simulink model "EmfObserver"  (R2026b)
settings: Solver=VariableStepAuto
undefined symbols (not defined in the file or in its folder): emfCfg, pllCfg
libraries: AngleTracking x2
settings Model: Creator=24322  LastModifiedBy=24322

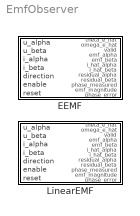
== system EmfObserver ==
  EEMF : Subsystem  mask{cfg=emfCfg, trackerCfg=pllCfg}
      mask prompts: cfg "Observer configuration"; trackerCfg "PLL configuration"
  LinearEMF : Subsystem  mask{cfg=emfCfg, trackerCfg=pllCfg}
      mask prompts: cfg "Observer configuration"; trackerCfg "PLL configuration"

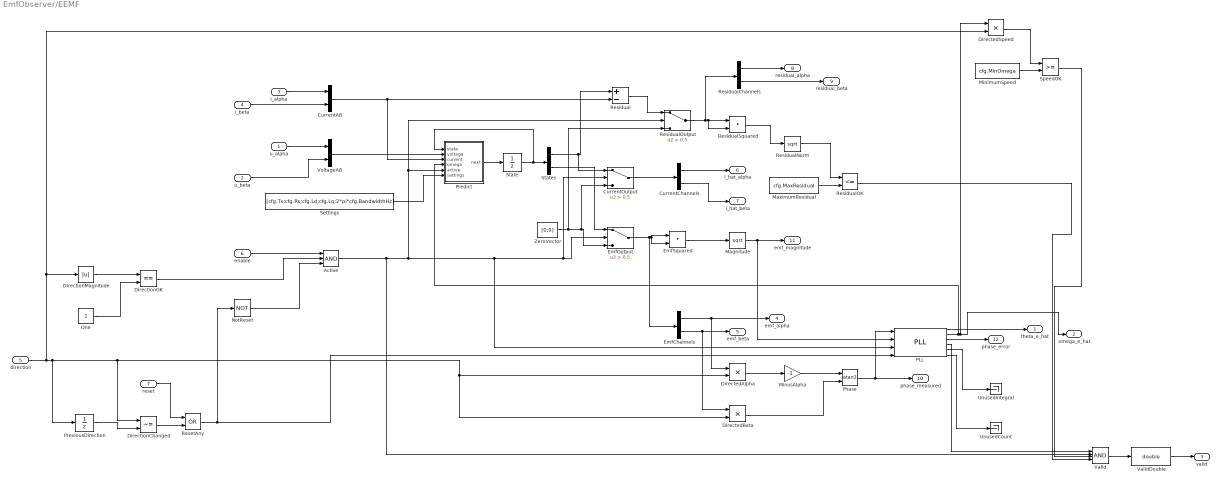
== system EmfObserver/EEMF ==
  u_alpha : Inport  SampleTime=cfg.Ts
  u_beta : Inport  Port=2  SampleTime=cfg.Ts
  i_alpha : Inport  Port=3  SampleTime=cfg.Ts
  i_beta : Inport  Port=4  SampleTime=cfg.Ts
  direction : Inport  Port=5  SampleTime=cfg.Ts
  enable : Inport  Port=6  SampleTime=cfg.Ts
  reset : Inport  Port=7  SampleTime=cfg.Ts
  Active : Logic  Inputs=3  IconShape=distinctive  AllPortsSameDT=off  OutDataTypeStr=boolean
  CurrentAB : Mux  Inputs=2
  CurrentChannels : Demux  Outputs=2
  CurrentOutput : Switch  Criteria=u2 > Threshold  Threshold=0.5  SaturateOnIntegerOverflow=off  InputSameDT=off
  DirectedAlpha : Product  Inputs=**
  DirectedBeta : Product  Inputs=**
  DirectedSpeed : Product  Inputs=**
  DirectionChanged : RelationalOperator  Operator=~=  OutDataTypeStr=boolean  RndMeth=Simplest  InputSameDT=off
  DirectionMagnitude : Abs  SaturateOnIntegerOverflow=off
  DirectionOK : RelationalOperator  Operator===  OutDataTypeStr=boolean  RndMeth=Simplest  InputSameDT=off
  EmfChannels : Demux  Outputs=2
  EmfOutput : Switch  Criteria=u2 > Threshold  Threshold=0.5  SaturateOnIntegerOverflow=off  InputSameDT=off
  EmfSquared : DotProduct  OutDataTypeStr=Inherit: Inherit via internal rule
  Magnitude : Sqrt
  MaximumResidual : Constant  Value=cfg.MaxResidual
  MinimumSpeed : Constant  Value=cfg.MinOmega
  MinusAlpha : Gain  Gain=-1
  NotReset : Logic  Operator=NOT  IconShape=distinctive  AllPortsSameDT=off  OutDataTypeStr=boolean
  One : Constant
  PLL : AngleTracking/PLL  pllCfg=trackerCfg
  Phase : Trigonometry  Operator=atan2
  Predict : MATLAB Function  TreatAsAtomicUnit=on
  PreviousDirection : UnitDelay  SampleTime=cfg.Ts
  ResetAny : Logic  Operator=OR  IconShape=distinctive  AllPortsSameDT=off  OutDataTypeStr=boolean
  Residual : Sum  Inputs=+-
  ResidualChannels : Demux  Outputs=2
  ResidualNorm : Sqrt
  ResidualOK : RelationalOperator  Operator=<=  OutDataTypeStr=boolean  RndMeth=Simplest  InputSameDT=off
  ResidualOutput : Switch  Criteria=u2 > Threshold  Threshold=0.5  SaturateOnIntegerOverflow=off  InputSameDT=off
  ResidualSquared : DotProduct  OutDataTypeStr=Inherit: Inherit via internal rule
  Settings : Constant  Value=[cfg.Ts;cfg.Rs;cfg.Ld;cfg.Lq;2*pi*cfg.BandwidthHz]
  SpeedOK : RelationalOperator  OutDataTypeStr=boolean  RndMeth=Simplest  InputSameDT=off
  State : UnitDelay  InitialCondition=zeros(4,1)  SampleTime=cfg.Ts
  States : Demux  Outputs=2
  UnusedCount : Terminator
  UnusedIntegral : Terminator
  Valid : Logic  Inputs=4  IconShape=distinctive  AllPortsSameDT=off  OutDataTypeStr=boolean
  ValidDouble : DataTypeConversion  OutDataTypeStr=double  SaturateOnIntegerOverflow=off  RndMeth=Floor
  VoltageAB : Mux  Inputs=2
  ZeroVector : Constant  Value=[0;0]
  theta_e_hat : Outport
  omega_e_hat : Outport  Port=2
  valid : Outport  Port=3
  emf_alpha : Outport  Port=4
  emf_beta : Outport  Port=5
  i_hat_alpha : Outport  Port=6
  i_hat_beta : Outport  Port=7
  residual_alpha : Outport  Port=8
  residual_beta : Outport  Port=9
  phase_measured : Outport  Port=10
  emf_magnitude : Outport  Port=11
  phase_error : Outport  Port=12
  wires:
  ResidualChannels/2 -> residual_beta/1
  CurrentChannels/2 -> i_hat_beta/1
  ResidualChannels/1 -> residual_alpha/1
  CurrentChannels/1 -> i_hat_alpha/1
  PLL/6 -> UnusedCount/1
  PLL/5 -> UnusedIntegral/1
  PLL/4 -> Valid/1
  PLL/3 -> phase_error/1
  PLL/1 -> theta_e_hat/1
  EmfChannels/2 -> emf_beta/1, DirectedBeta/1
  EmfChannels/1 -> emf_alpha/1, DirectedAlpha/1
  States/2 -> EmfOutput/1
  States/1 -> CurrentOutput/1, Residual/1
  Predict/1(next) -> State/1
  Settings/1 -> Predict/6(settings)
  PLL/2 -> omega_e_hat/1, DirectedSpeed/1, Predict/4(omega)
  VoltageAB/1 -> Predict/2(voltage)
  ValidDouble/1 -> valid/1
  Valid/1 -> ValidDouble/1
  ResidualOK/1 -> Valid/4
  SpeedOK/1 -> Valid/3
  MinimumSpeed/1 -> SpeedOK/2
  DirectedSpeed/1 -> SpeedOK/1
  Magnitude/1 -> PLL/2, emf_magnitude/1
  Phase/1 -> PLL/1, phase_measured/1
  DirectedBeta/1 -> Phase/2
  MinusAlpha/1 -> Phase/1
  DirectedAlpha/1 -> MinusAlpha/1
  EmfSquared/1 -> Magnitude/1
  MaximumResidual/1 -> ResidualOK/2
  ResidualNorm/1 -> ResidualOK/1
  ResidualSquared/1 -> ResidualNorm/1
  ZeroVector/1 -> CurrentOutput/3, EmfOutput/3, ResidualOutput/3
  Active/1 -> CurrentOutput/2, EmfOutput/2, PLL/3, ResidualOutput/2, Predict/5(active), Valid/2
  Residual/1 -> ResidualOutput/1
  CurrentAB/1 -> Residual/2, Predict/3(current)
  ResidualOutput/1 -> ResidualSquared/1, ResidualSquared/2, ResidualChannels/1
  EmfOutput/1 -> EmfSquared/1, EmfSquared/2, EmfChannels/1
  CurrentOutput/1 -> CurrentChannels/1
  State/1 -> States/1, Predict/1(state)
  NotReset/1 -> Active/3
  DirectionOK/1 -> Active/2
  enable/1 -> Active/1
  ResetAny/1 -> NotReset/1, PLL/4
  DirectionChanged/1 -> ResetAny/2
  reset/1 -> ResetAny/1
  PreviousDirection/1 -> DirectionChanged/2
  One/1 -> DirectionOK/2
  DirectionMagnitude/1 -> DirectionOK/1
  direction/1 -> DirectedAlpha/2, DirectedBeta/2, DirectionChanged/1, PreviousDirection/1, DirectionMagnitude/1, DirectedSpeed/2
  i_beta/1 -> CurrentAB/2
  i_alpha/1 -> CurrentAB/1
  u_beta/1 -> VoltageAB/2
  u_alpha/1 -> VoltageAB/1

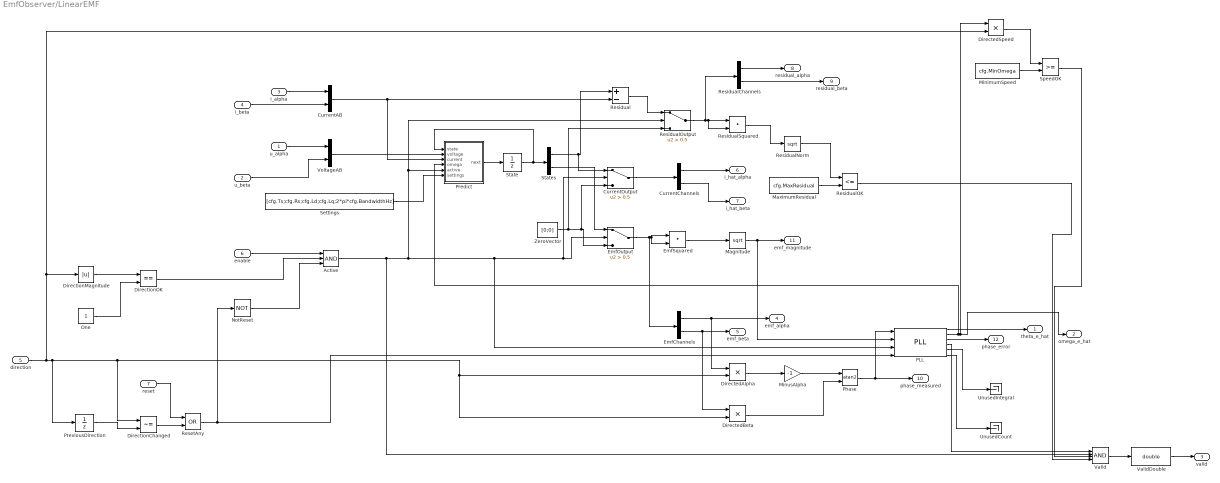
== system EmfObserver/LinearEMF ==
  u_alpha : Inport  SampleTime=cfg.Ts
  u_beta : Inport  Port=2  SampleTime=cfg.Ts
  i_alpha : Inport  Port=3  SampleTime=cfg.Ts
  i_beta : Inport  Port=4  SampleTime=cfg.Ts
  direction : Inport  Port=5  SampleTime=cfg.Ts
  enable : Inport  Port=6  SampleTime=cfg.Ts
  reset : Inport  Port=7  SampleTime=cfg.Ts
  Active : Logic  Inputs=3  IconShape=distinctive  AllPortsSameDT=off  OutDataTypeStr=boolean
  CurrentAB : Mux  Inputs=2
  CurrentChannels : Demux  Outputs=2
  CurrentOutput : Switch  Criteria=u2 > Threshold  Threshold=0.5  SaturateOnIntegerOverflow=off  InputSameDT=off
  DirectedAlpha : Product  Inputs=**
  DirectedBeta : Product  Inputs=**
  DirectedSpeed : Product  Inputs=**
  DirectionChanged : RelationalOperator  Operator=~=  OutDataTypeStr=boolean  RndMeth=Simplest  InputSameDT=off
  DirectionMagnitude : Abs  SaturateOnIntegerOverflow=off
  DirectionOK : RelationalOperator  Operator===  OutDataTypeStr=boolean  RndMeth=Simplest  InputSameDT=off
  EmfChannels : Demux  Outputs=2
  EmfOutput : Switch  Criteria=u2 > Threshold  Threshold=0.5  SaturateOnIntegerOverflow=off  InputSameDT=off
  EmfSquared : DotProduct  OutDataTypeStr=Inherit: Inherit via internal rule
  Magnitude : Sqrt
  MaximumResidual : Constant  Value=cfg.MaxResidual
  MinimumSpeed : Constant  Value=cfg.MinOmega
  MinusAlpha : Gain  Gain=-1
  NotReset : Logic  Operator=NOT  IconShape=distinctive  AllPortsSameDT=off  OutDataTypeStr=boolean
  One : Constant
  PLL : AngleTracking/PLL  pllCfg=trackerCfg
  Phase : Trigonometry  Operator=atan2
  Predict : MATLAB Function  TreatAsAtomicUnit=on
  PreviousDirection : UnitDelay  SampleTime=cfg.Ts
  ResetAny : Logic  Operator=OR  IconShape=distinctive  AllPortsSameDT=off  OutDataTypeStr=boolean
  Residual : Sum  Inputs=+-
  ResidualChannels : Demux  Outputs=2
  ResidualNorm : Sqrt
  ResidualOK : RelationalOperator  Operator=<=  OutDataTypeStr=boolean  RndMeth=Simplest  InputSameDT=off
  ResidualOutput : Switch  Criteria=u2 > Threshold  Threshold=0.5  SaturateOnIntegerOverflow=off  InputSameDT=off
  ResidualSquared : DotProduct  OutDataTypeStr=Inherit: Inherit via internal rule
  Settings : Constant  Value=[cfg.Ts;cfg.Rs;cfg.Ld;cfg.Lq;2*pi*cfg.BandwidthHz]
  SpeedOK : RelationalOperator  OutDataTypeStr=boolean  RndMeth=Simplest  InputSameDT=off
  State : UnitDelay  InitialCondition=zeros(4,1)  SampleTime=cfg.Ts
  States : Demux  Outputs=2
  UnusedCount : Terminator
  UnusedIntegral : Terminator
  Valid : Logic  Inputs=4  IconShape=distinctive  AllPortsSameDT=off  OutDataTypeStr=boolean
  ValidDouble : DataTypeConversion  OutDataTypeStr=double  SaturateOnIntegerOverflow=off  RndMeth=Floor
  VoltageAB : Mux  Inputs=2
  ZeroVector : Constant  Value=[0;0]
  theta_e_hat : Outport
  omega_e_hat : Outport  Port=2
  valid : Outport  Port=3
  emf_alpha : Outport  Port=4
  emf_beta : Outport  Port=5
  i_hat_alpha : Outport  Port=6
  i_hat_beta : Outport  Port=7
  residual_alpha : Outport  Port=8
  residual_beta : Outport  Port=9
  phase_measured : Outport  Port=10
  emf_magnitude : Outport  Port=11
  phase_error : Outport  Port=12
  wires:
  ResidualChannels/2 -> residual_beta/1
  CurrentChannels/2 -> i_hat_beta/1
  ResidualChannels/1 -> residual_alpha/1
  CurrentChannels/1 -> i_hat_alpha/1
  PLL/6 -> UnusedCount/1
  PLL/5 -> UnusedIntegral/1
  PLL/4 -> Valid/1
  PLL/3 -> phase_error/1
  PLL/1 -> theta_e_hat/1
  EmfChannels/2 -> emf_beta/1, DirectedBeta/1
  EmfChannels/1 -> emf_alpha/1, DirectedAlpha/1
  States/2 -> EmfOutput/1
  States/1 -> CurrentOutput/1, Residual/1
  Predict/1(next) -> State/1
  Settings/1 -> Predict/6(settings)
  PLL/2 -> omega_e_hat/1, DirectedSpeed/1, Predict/4(omega)
  VoltageAB/1 -> Predict/2(voltage)
  ValidDouble/1 -> valid/1
  Valid/1 -> ValidDouble/1
  ResidualOK/1 -> Valid/4
  SpeedOK/1 -> Valid/3
  MinimumSpeed/1 -> SpeedOK/2
  DirectedSpeed/1 -> SpeedOK/1
  Magnitude/1 -> PLL/2, emf_magnitude/1
  Phase/1 -> PLL/1, phase_measured/1
  DirectedBeta/1 -> Phase/2
  MinusAlpha/1 -> Phase/1
  DirectedAlpha/1 -> MinusAlpha/1
  EmfSquared/1 -> Magnitude/1
  MaximumResidual/1 -> ResidualOK/2
  ResidualNorm/1 -> ResidualOK/1
  ResidualSquared/1 -> ResidualNorm/1
  ZeroVector/1 -> CurrentOutput/3, EmfOutput/3, ResidualOutput/3
  Active/1 -> CurrentOutput/2, EmfOutput/2, PLL/3, ResidualOutput/2, Predict/5(active), Valid/2
  Residual/1 -> ResidualOutput/1
  CurrentAB/1 -> Residual/2, Predict/3(current)
  ResidualOutput/1 -> ResidualSquared/1, ResidualSquared/2, ResidualChannels/1
  EmfOutput/1 -> EmfSquared/1, EmfSquared/2, EmfChannels/1
  CurrentOutput/1 -> CurrentChannels/1
  State/1 -> States/1, Predict/1(state)
  NotReset/1 -> Active/3
  DirectionOK/1 -> Active/2
  enable/1 -> Active/1
  ResetAny/1 -> NotReset/1, PLL/4
  DirectionChanged/1 -> ResetAny/2
  reset/1 -> ResetAny/1
  PreviousDirection/1 -> DirectionChanged/2
  One/1 -> DirectionOK/2
  DirectionMagnitude/1 -> DirectionOK/1
  direction/1 -> DirectedAlpha/2, DirectedBeta/2, DirectionChanged/1, PreviousDirection/1, DirectionMagnitude/1, DirectedSpeed/2
  i_beta/1 -> CurrentAB/2
  i_alpha/1 -> CurrentAB/1
  u_beta/1 -> VoltageAB/2
  u_alpha/1 -> VoltageAB/1

== matlab function EmfObserver/EEMF/Predict ==
  data: state input; next output; voltage input; current input; omega input; active input; settings input
function next=emf_predict(state,voltage,current,omega,active,settings)
%EMF_PREDICT Full-order current/extended-EMF observer, forward Euler.
% state=[i_hat_alpha;i_hat_beta;e_hat_alpha;e_hat_beta].
% current[k] and interval-start voltage[k] update state[k+1].
% settings=[Ts;Rs;Ld;Lq;observer_pole_rad_s]. No true angle/speed input.
%#codegen
next=zeros(4,1,'like',state);
if ~active,return;end
step=settings(1);resistance=settings(2);ld=settings(3);lq=settings(4);pole=settings(5);
ihat=state(1:2);emf=state(3:4);innovation=current-ihat;
jcurrent=[-ihat(2);ihat(1)];jemf=[-emf(2);emf(1)];
l1=2*pole-resistance/ld;l2=-ld*pole*pole;
di=(-resistance*ihat+omega*(ld-lq)*jcurrent-emf+voltage)/ld+l1*innovation;
de=omega*jemf+l2*innovation;
next(1:2)=ihat+step*di;next(3:4)=emf+step*de;
end

== matlab function EmfObserver/LinearEMF/Predict ==
  data: state input; next output; voltage input; current input; omega input; active input; settings input
function next=emf_predict(state,voltage,current,omega,active,settings)
%EMF_PREDICT Full-order current/extended-EMF observer, forward Euler.
% state=[i_hat_alpha;i_hat_beta;e_hat_alpha;e_hat_beta].
% current[k] and interval-start voltage[k] update state[k+1].
% settings=[Ts;Rs;Ld;Lq;observer_pole_rad_s]. No true angle/speed input.
%#codegen
next=zeros(4,1,'like',state);
if ~active,return;end
step=settings(1);resistance=settings(2);ld=settings(3);lq=settings(4);pole=settings(5);
ihat=state(1:2);emf=state(3:4);innovation=current-ihat;
jcurrent=[-ihat(2);ihat(1)];jemf=[-emf(2);emf(1)];
l1=2*pole-resistance/ld;l2=-ld*pole*pole;
di=(-resistance*ihat+omega*(ld-lq)*jcurrent-emf+voltage)/ld+l1*innovation;
de=omega*jemf+l2*innovation;
next(1:2)=ihat+step*di;next(3:4)=emf+step*de;
end
